simulink model "sm_robot_run_4legs"  (R2025a)
settings: Solver=ode15s  StartTime=0.0  StopTime=t_final  MaxStep=0.01  RelTol=1e-3  AbsTol=1e-4  EnableMultiTasking=on
InitFcn:
  | d2r = pi/180;
  | r2d = 180/pi;
  | if (~exist('t_final'))
  |   sm_robot_run_4legs_param_def_load(bdroot)
  | end
values from neighbouring files (symbols this model uses):
  N = 100    [Extr_Data_Cam_Roller_Curve.m]
  s = sin(q)    [Extr_Data_Cam_Roller_Curve.m]
undefined symbols (not defined in the file or in its folder): Extr_Data_Mesh, l1, L_back, L_stance, M, T_cg, th2, u0, X, Y, Z
libraries: sm_lib x32, nesl_utility x10, fl_lib x5, sm_robot_run_4legs_lib x4, batteryecm_lib x1
(part 1 of 2)
CloseFcn:
  | try,close(h1_sm_robot_run_4legs),end
  | clear h1_sm_robot_run_4legs
  | try,close(h2_sm_robot_run_4legs),end
  | clear h2_sm_robot_run_4legs
  | try,close(h3_sm_robot_run_4legs),end
  | clear h3_sm_robot_run_4legs
  | try,close(h4_sm_robot_run_4legs),end
  | clear h4_sm_robot_run_4legs
  | 
  | 
  | clear simlog_sm_robot_run_4legs
  | clear logsout_sm_robot_run_4legs
Description:
  | Mechatronic Running Robot
  | 
  | Copyright 2012-2025 The MathWorks, Inc.
settings Model: Creator=rhyde  LastModifiedBy=smiller
settings SolverCC: AutoScaleAbsTol=off  MaxConsecutiveZCs=10000  AlgebraicLoopSolver=TrustRegion
settings DataIOCC: MaxDataPoints=10000  SaveFinalState=on  SaveFormat=Array  SignalLoggingSaveFormat=ModelDataLogs  SaveState=on  ReturnWorkspaceOutputs=off  SignalLoggingName=logsout_sm_robot_run_4legs  OutputTimes=[0:0.01:t_final]
settings OptimizationCC: ReuseModelBlockBuffer=off  ExpressionDepthLimit=2147483647.0  InitFltsAndDblsToZero=on  LifeSpan=inf
settings DebuggingCC: SaveWithParameterizedLinksMsg=none  UnderspecifiedInitializationDetection=Classic  MergeDetectMultiDrivingBlocksExec=none  SignalResolutionControl=TryResolveAllWithWarning  SolverPrmCheckMsg=warning  MultiTaskDSMMsg=warning  MultiTaskCondExecSysMsg=none  FcnCallInpInsideContextMsg=warning  UnconnectedInputMsg=warning  UnconnectedOutputMsg=warning  UnconnectedLineMsg=warning  StateNameClashWarn=warning  PregeneratedLibrarySubsystemCodeDiagnostic=none  SFUnexpectedBacktrackingDiag=warning  SFNoUnconditionalDefaultTransitionDiag=warning  SFExecutionAtInitializationDiag=none  ArithmeticOperatorsInVariantConditions=warning
settings HardwareCC: ProdBitPerPointer=32.0  ProdBitPerSizeT=32.0  ProdBitPerPtrDiffT=32.0  ProdLargestAtomicFloat=None  ProdIntDivRoundTo=Undefined  ProdEndianess=Unspecified  ProdWordSize=32.0  ProdHWDeviceType=32-bit Generic
settings ModelReferenceCC: EnableRefExpFcnMdlSchedulingChecks=on  PropagateSignalLabelsOutOfModel=off
settings SFSimCC: SimUseLocalCustomCode=off  SimParseCustomCode=off  CustomCodeUndefinedFunction=UseInterfaceOnly
settings RTWCC: RTWUseLocalCustomCode=off  GPUComputeCapability=3.5  DLArmComputeVersion=19.05
settings CodeAppCC: StateflowObjectComments=on
settings GRTTargetCC: TargetFcnLib=ansi_tfl_tmw.mat  TargetLangStandard=C89/C90 (ANSI)  CombineOutputUpdateFcns=off  GRTInterface=on
settings ConfigComp: CovMetricSettings=dw  CovSaveCumulativeToWorkspaceVar=on  CovSaveSingleToWorkspaceVar=on  CovExternalEMLEnable=off
settings SimscapeCC: SimscapeNormalizeSystem=off  SimscapeLogType=all  SimscapeLogSimulationStatistics=on  SimscapeLogName=simlog_sm_robot_run_4legs  SimscapeLogDataHistory=50000.0
settings ConfigurationSet: Description=SimMechanics 2G
settings DiagnosticsConfigSet: SimMechanicsUnconnectedFramePorts=none  SimMechanicsRigidlyBoundBlock=none
settings ExplorerConfigSet: InternalSimMechanicsExplorerSettings="<ExplorerConfiguration><canonicalview>default</canonicalview><AnimationSetting><BasePlaybackSpeed>1.0</BasePlaybackSpeed><PlaybackSpeedFactor>0.5</PlaybackSpeedFactor></AnimationSetting><TilePanel><TileInfo><Tiles Columns=\"1\" Count=\"1\" Rows=\"1\"><Column Weight=\"1\"/><Row Weight=\"1\"/><Tile Height=\"1\" Width=\"1\" X=\"0\" Y=\"0\"/></Tiles></TileInfo><SceneInfo><SceneViewer><BGColor><R>1</R><G>1</G><B>1</B></BGColor><Camera><DoPerspective>on</DoPerspective><Position><X>9.65055700274290018</X><Y>0.935000000000000053</Y><Z>1.00000000000000089</Z></Position><Center><X>8.79768847079045635</X><Y>0.76135182233306975</Y><Z>0.507596123493896711</Z></Center><Up><X>0</X><Y>1</Y><Z>0</Z></Up><ViewLimDist>1</ViewLimDist><YLim>0.466307658154998583</YLim><XLim>0.552660928183702049</XLim></Camera></SceneViewer></SceneInfo></TilePanel><MechEditorPanel><Cameras><Camera><Id>Camera1</Id><Value><Name>Body</Name><NativeCamera><PositionTrackingFeature>Body_Constraint.Camera.Transform_Camera.F</PositionTrackingFeature><CenterTrackingFeature>Body_Constraint.World_Frame.W</CenterTrackingFeature><UpVectorTrackingFeature>Body_Constraint.World_Frame.W</UpVectorTrackingFeature><CenterTrackingOrigin>off</CenterTrackingOrigin><CenterTrackingDirection>-Z</CenterTrackingDirection><UpVectorTrackingDirection>+Y</UpVectorTrackingDirection></NativeCamera></Value></Camera><Camera><Id>Camera2</Id><Value><Name>Body_Iso</Name><NativeCamera><PositionTrackingFeature>Body_Constraint.Camera.Transform_Camera_BodyIso.F</PositionTrackingFeature><CenterTrackingFeature>Body_Constraint.Camera.Transform_Camera_BodyIso_Aim.F</CenterTrackingFeature><UpVectorTrackingFeature>Body_Constraint.World_Frame.W</UpVectorTrackingFeature><CenterTrackingOrigin>off</CenterTrackingOrigin><CenterTrackingDirection>-Z</CenterTrackingDirection><UpVectorTrackingDirection>+Y</UpVectorTrackingDirection></NativeCamera></Value></Camera></Cameras><GfxPanelCameraMap><MapElement CameraMLId=\"Camera2\" GfxPanelIndex=\"0\"/></GfxPanelCameraMap><VideoCreator><PlaybackSpeedRatio>1.0</PlaybackSpeedRatio><FrameRate>30</FrameRate><VideoFormat>Motion JPEG AVI</VideoFormat><FrameSize>auto</FrameSize></VideoCreator></MechEditorPanel></ExplorerConfiguration>"

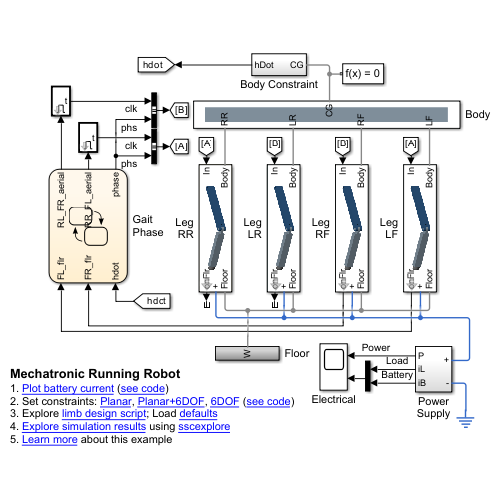
[thumbnail: Simulink's stored preview of the top-level diagram]
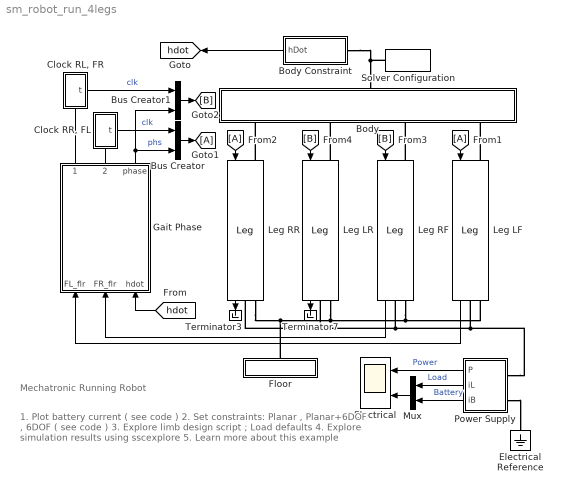
== system sm_robot_run_4legs ==
  note: Mechatronic Running Robot
  note: 1. Plot battery current ( see code )
      | 2. Set constraints: Planar , Planar+6DOF , 6DOF ( see code )
      | 3. Explore limb design script ; Load defaults
      | 4. Explore simulation results using sscexplore
      | 5. Learn more about this example
  Body : Subsystem  Tag=CustomStyle
      mask Display: image('sm_robot_run_body_IMAGE.png')
  Body Constraint : Subsystem
  Bus Creator : BusCreator  Inputs=2
  Bus Creator1 : BusCreator  Inputs=2
  "Clock RL, FR" : Subsystem  TreatAsAtomicUnit=on  mask{t0=0}
      mask prompts: t0 "Initial local time"
  "Clock RR, FL" : Subsystem  TreatAsAtomicUnit=on  mask{t0=3*T_cg/4}
      mask prompts: t0 "Initial local time"
  Electrical : Scope  NumInputPorts=2
      settings: ActiveDisplayYMinimum=-181.58066  ActiveDisplayYMaximum=525.06229
  Electrical Reference : fl_lib/Electrical/Electrical Elements/Electrical Reference
  Floor : Subsystem
  From1 : From
  From2 : From
  Gait Phase : Stateflow chart  Tag=PublishSubsystem  TreatAsAtomicUnit=on
  Goto1 : Goto
  Leg LF : sm_robot_run_4legs_lib/Leg  Tag=PublishSubsystemCustomStyle  leg_type=Front Left  leg_width=0.1*l1  th1_0=d2r*u_th(find(t_th > 3*T_cg/4,1))  th2_0=-50*d2r+th2  th1_dot_0=-d2r*u_w(find(t_th > 3*T_cg/4,1))  x0=L_back  popup_contact_model=Planar
  Leg LR : sm_robot_run_4legs_lib/Leg  Tag=CustomStyle  leg_type=Rear Left  leg_width=0.1*l1  th1_0=th1_0  th2_0=th2_0  th1_dot_0=u0/L_stance  x0=0  popup_contact_model=Planar
  Leg RF : sm_robot_run_4legs_lib/Leg  Tag=CustomStyle  leg_type=Front Right  leg_width=0.1*l1  th1_0=th1_0  th2_0=th2_0  th1_dot_0=u0/L_stance  x0=L_back  popup_contact_model=Planar
  Leg RR : sm_robot_run_4legs_lib/Leg  Tag=CustomStyle  leg_type=Rear Right  leg_width=0.1*l1  th1_0=d2r*u_th(find(t_th > 3*T_cg/4,1))  th2_0=-50*d2r+th2  th1_dot_0=-d2r*u_w(find(t_th > 3*T_cg/4,1))  x0=0  popup_contact_model=Planar
  Mux : Mux  Inputs=2
  Power Supply : Subsystem  Tag=PublishSubsystem
  Solver Configuration : nesl_utility/Solver Configuration  PhysicalDomain=network_engine_domain  SubClassName=solver  LeftPortType=input  RightPortType=generic  Tones=[]  Harmonics=[]  SimulateNoise=off  Profile=off  UseLocalSampling=off  EnableSwitchedLinearOptims=on  FrequencyDomain=off  UseCCode=off  RelTol=0.001  AbsTol=1e-06  MinStep=1e-09  ToWorkspace=off  RevertToSquareIcSolve=off  NumHomotopyIterations=100  PhasorMode=off  PhasorModeNumHarmonics=1  ConsistencySolver=NEWTON_FTOL  IndexReductionMethod=DerivativeReplacement  DoDC=off  ResidualTolerance=1e-9  ConsistencyTolSource=GLOBAL  ConsistencyAbsTol=0.001  ConsistencyRelTol=0.001  ConsistencyTolFactor=0.001  UseLocalSolver=off  LocalSolverChoice=NE_BACKWARD_EULER_ADVANCER  ResolveIndetEquations=on  FunctionEvalNumThread=1  LocalSolverSampleTime=.001  DoFixedCost=off  MaxNonlinIter=12  MaxModeIter=2  ComputeImpulses=off  ImpulseIterations=2  LinearAlgebra=Sparse  LinearAlgebraNumThread=0  EquationFormulation=NE_TIME_EF  DelaysMemoryBudget=1024  AutomaticFiltering=on  FilteringTimeConstant=0.001  PartitionStorageMethod=AS_NEEDED  PartitionMemoryBudget=1024  PartitionMethod=FAST  MultibodyUseLocalSolver=off  MultibodyLocalSolverChoice=ODE1  MultibodyLocalSolverSampleTime=0.001
  Terminator3 : Terminator
  Terminator7 : Terminator
  tag scope: hdot=global
  wires:
  [hdot] -> Gait Phase/3(hdot)
  Leg RR/1 -> Terminator3/1
  Leg LF/1 -> Gait Phase/1(FL_flr)
  Leg LR/1 -> Terminator7/1
  Gait Phase/1(RL_FR_aerial) -> "Clock RL, FR"/Enable
  Gait Phase/2(RR_FL_aerial) -> "Clock RR, FL"/Enable
  "Clock RR, FL"/1(t) -> Bus Creator/1  "clk"
  Leg RF/1 -> Gait Phase/2(FR_flr)
  Power Supply/2(iL) -> Mux/1  "Load"
  Power Supply/1(P) -> Electrical/1  "Power"
  Bus Creator/1 -> Goto1/1
  Bus Creator1/1 -> [B]
  "Clock RL, FR"/1(t) -> Bus Creator1/1  "clk"
  Gait Phase/3(phase) -> Bus Creator1/2, Bus Creator/2  "phs"
  From1/1 -> Leg LF/1
  From2/1 -> Leg RR/1
  [B] -> Leg RF/1
  [B] -> Leg LR/1
  Body Constraint/1(hDot) -> [hdot]
  Mux/1 -> Electrical/2
  Power Supply/3(iB) -> Mux/2  "Battery"
  connections:
  Body Constraint/LConn1 -- Solver Configuration/RConn1 -- Body/RConn1
  Power Supply/LConn2 -- Electrical Reference/LConn1
  Power Supply/LConn1 -- Leg RR/RConn1 -- Leg LR/RConn1 -- Leg RF/RConn1 -- Leg LF/RConn1
  Leg LF/LConn1 -- Body/LConn4
  Leg RF/LConn1 -- Body/LConn3
  Leg LR/LConn1 -- Body/LConn2
  Leg RR/LConn1 -- Body/LConn1
  Floor/RConn1 -- Leg LF/RConn2 -- Leg RF/RConn2 -- Leg LR/RConn2 -- Leg RR/RConn2

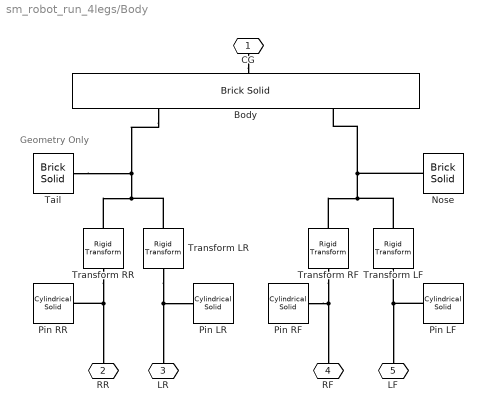
== system sm_robot_run_4legs/Body ==
  note: Geometry Only
  Body : sm_lib/Body Elements/Brick Solid  BrickDimensions=[1 0.1 0.1]*L_back  BrickDimensionsUnits=m  ExportEntireGeometry=off  InertiaType=Custom  BasedOnType=Density  Density=1000  DensityUnits=kg/m^3  Mass=M*2  MassUnits=kg  CenterOfMass=[0 0 0]  CenterOfMassUnits=m  MomentsOfInertia=[1 1 1]*(1/12)*2*M*L_back^2*100  MomentsOfInertiaUnits=kg*m^2  ProductsOfInertia=[1 1 1]*0  ProductsOfInertiaUnits=kg*m^2  GraphicType=FromGeometry  MarkerShape=Sphere  MarkerSize=10  GraphicVisPropType=SimpleVisualProperties  GraphicDiffuseColor=[164 184 200]/255  GraphicOpacity=1.0  GraphicSpecularColor=[0.5 0.5 0.5 1.0]  GraphicAmbientColor=[0.15 0.15 0.15 1.0]  GraphicEmissiveColor=[0.0 0.0 0.0 1.0]  GraphicShininess=75  DoExposeReferenceFrame=on  SerializedFrames=<Frames><Frame><Id>Frame1</Id><Value><Name>B</Name><Origin><Source>GeometricFeature</Source><FeatureName>-x surface</FeatureName></Origin><PrimaryAxis><DefinedDirection>+Z</DefinedDirection><Source>ReferenceFrame</Source><SourceDirection>+Z</SourceDirection><FeatureName></FeatureName></PrimaryAxis><SecondaryAxis><DefinedDirection>+X</DefinedDirection><Source>ReferenceFrame</Source><SourceDirection>+X</SourceDirection><FeatureName></FeatureName></SecondaryAxis></Value></Frame><Frame><Id>Frame2</Id><Value><Name>F</Name><Origin><Source>GeometricFeature</Source><FeatureName>+x surface</FeatureName></Origin><PrimaryAxis><DefinedDirection>+Z</DefinedDirection><Source>ReferenceFrame</Source><SourceDirection>+Z</SourceDirection><FeatureName></FeatureName></PrimaryAxis><SecondaryAxis><DefinedDirection>+X</DefinedDirection><Source>ReferenceFrame</Source><SourceDirection>+X</SourceDirection><FeatureName></FeatureName></SecondaryAxis></Value></Frame></Frames>
  Nose : sm_lib/Body Elements/Brick Solid  BrickDimensions=[0.05 0.1 0.1]*L_back  BrickDimensionsUnits=m  ExportEntireGeometry=off  InertiaType=CalculateFromGeometry  BasedOnType=Density  Density=0  DensityUnits=kg/m^3  Mass=1  MassUnits=kg  CenterOfMass=[0 0 0]  CenterOfMassUnits=m  MomentsOfInertia=[1 1 1]  MomentsOfInertiaUnits=kg*m^2  ProductsOfInertia=[1 1 1]  ProductsOfInertiaUnits=kg*m^2  GraphicType=FromGeometry  MarkerShape=Sphere  MarkerSize=10  GraphicVisPropType=SimpleVisualProperties  GraphicDiffuseColor=[164 184 200]/255  GraphicOpacity=1.0  GraphicSpecularColor=[0.5 0.5 0.5 1.0]  GraphicAmbientColor=[0.15 0.15 0.15 1.0]  GraphicEmissiveColor=[0.0 0.0 0.0 1.0]  GraphicShininess=75  DoExposeReferenceFrame=off  SerializedFrames=<Frames><Frame><Id>Frame1</Id><Value><Name>B</Name><Origin><Source>GeometricFeature</Source><FeatureName>-x surface</FeatureName></Origin><PrimaryAxis><DefinedDirection>+Z</DefinedDirection><Source>ReferenceFrame</Source><SourceDirection>+Z</SourceDirection><FeatureName></FeatureName></PrimaryAxis><SecondaryAxis><DefinedDirection>+X</DefinedDirection><Source>ReferenceFrame</Source><SourceDirection>+X</SourceDirection><FeatureName></FeatureName></SecondaryAxis></Value></Frame></Frames>
  Pin LF : sm_lib/Body Elements/Cylindrical Solid  CylinderRadius=0.025*l1  CylinderRadiusUnits=m  CylinderLength=0.1*l1  CylinderLengthUnits=m  ExportEntireGeometry=off  InertiaType=CalculateFromGeometry  BasedOnType=Density  Density=0  DensityUnits=kg/m^3  Mass=1  MassUnits=kg  CenterOfMass=[0 0 0]  CenterOfMassUnits=m  MomentsOfInertia=[1 1 1]  MomentsOfInertiaUnits=kg*m^2  ProductsOfInertia=[1 1 1]  ProductsOfInertiaUnits=kg*m^2  GraphicType=FromGeometry  MarkerShape=Sphere  MarkerSize=10  GraphicVisPropType=SimpleVisualProperties  GraphicDiffuseColor=[164 184 200]/255  GraphicOpacity=1.0  GraphicSpecularColor=[0.5 0.5 0.5 1.0]  GraphicAmbientColor=[0.15 0.15 0.15 1.0]  GraphicEmissiveColor=[0.0 0.0 0.0 1.0]  GraphicShininess=75  DoExposeReferenceFrame=off  SerializedFrames=<Frames><Frame><Id>Frame1</Id><Value><Name>F</Name><Origin><Source>GeometricFeature</Source><FeatureName>top surface</FeatureName></Origin><PrimaryAxis><DefinedDirection>+Z</DefinedDirection><Source>ReferenceFrame</Source><SourceDirection>+Z</SourceDirection><FeatureName></FeatureName></PrimaryAxis><SecondaryAxis><DefinedDirection>+X</DefinedDirection><Source>ReferenceFrame</Source><SourceDirection>+X</SourceDirection><FeatureName></FeatureName></SecondaryAxis></Value></Frame><Frame><Id>Frame2</Id><Value><Name>B</Name><Origin><Source>GeometricFeature</Source><FeatureName>bottom surface</FeatureName></Origin><PrimaryAxis><DefinedDirection>+Z</DefinedDirection><Source>ReferenceFrame</Source><SourceDirection>+Z</SourceDirection><FeatureName></FeatureName></PrimaryAxis><SecondaryAxis><DefinedDirection>+X</DefinedDirection><Source>ReferenceFrame</Source><SourceDirection>+X</SourceDirection><FeatureName></FeatureName></SecondaryAxis></Value></Frame></Frames>
  Pin LR : sm_lib/Body Elements/Cylindrical Solid  CylinderRadius=0.025*l1  CylinderRadiusUnits=m  CylinderLength=0.1*l1  CylinderLengthUnits=m  ExportEntireGeometry=off  InertiaType=CalculateFromGeometry  BasedOnType=Density  Density=0  DensityUnits=kg/m^3  Mass=1  MassUnits=kg  CenterOfMass=[0 0 0]  CenterOfMassUnits=m  MomentsOfInertia=[1 1 1]  MomentsOfInertiaUnits=kg*m^2  ProductsOfInertia=[1 1 1]  ProductsOfInertiaUnits=kg*m^2  GraphicType=FromGeometry  MarkerShape=Sphere  MarkerSize=10  GraphicVisPropType=SimpleVisualProperties  GraphicDiffuseColor=[164 184 200]/255  GraphicOpacity=1.0  GraphicSpecularColor=[0.5 0.5 0.5 1.0]  GraphicAmbientColor=[0.15 0.15 0.15 1.0]  GraphicEmissiveColor=[0.0 0.0 0.0 1.0]  GraphicShininess=75  DoExposeReferenceFrame=off  SerializedFrames=<Frames><Frame><Id>Frame1</Id><Value><Name>F</Name><Origin><Source>GeometricFeature</Source><FeatureName>top surface</FeatureName></Origin><PrimaryAxis><DefinedDirection>+Z</DefinedDirection><Source>ReferenceFrame</Source><SourceDirection>+Z</SourceDirection><FeatureName></FeatureName></PrimaryAxis><SecondaryAxis><DefinedDirection>+X</DefinedDirection><Source>ReferenceFrame</Source><SourceDirection>+X</SourceDirection><FeatureName></FeatureName></SecondaryAxis></Value></Frame><Frame><Id>Frame2</Id><Value><Name>B</Name><Origin><Source>GeometricFeature</Source><FeatureName>bottom surface</FeatureName></Origin><PrimaryAxis><DefinedDirection>+Z</DefinedDirection><Source>ReferenceFrame</Source><SourceDirection>+Z</SourceDirection><FeatureName></FeatureName></PrimaryAxis><SecondaryAxis><DefinedDirection>+X</DefinedDirection><Source>ReferenceFrame</Source><SourceDirection>+X</SourceDirection><FeatureName></FeatureName></SecondaryAxis></Value></Frame></Frames>
  Pin RF : sm_lib/Body Elements/Cylindrical Solid  CylinderRadius=0.025*l1  CylinderRadiusUnits=m  CylinderLength=0.1*l1  CylinderLengthUnits=m  ExportEntireGeometry=off  InertiaType=CalculateFromGeometry  BasedOnType=Density  Density=0  DensityUnits=kg/m^3  Mass=1  MassUnits=kg  CenterOfMass=[0 0 0]  CenterOfMassUnits=m  MomentsOfInertia=[1 1 1]  MomentsOfInertiaUnits=kg*m^2  ProductsOfInertia=[1 1 1]  ProductsOfInertiaUnits=kg*m^2  GraphicType=FromGeometry  MarkerShape=Sphere  MarkerSize=10  GraphicVisPropType=SimpleVisualProperties  GraphicDiffuseColor=[164 184 200]/255  GraphicOpacity=1.0  GraphicSpecularColor=[0.5 0.5 0.5 1.0]  GraphicAmbientColor=[0.15 0.15 0.15 1.0]  GraphicEmissiveColor=[0.0 0.0 0.0 1.0]  GraphicShininess=75  DoExposeReferenceFrame=off  SerializedFrames=<Frames><Frame><Id>Frame1</Id><Value><Name>F</Name><Origin><Source>GeometricFeature</Source><FeatureName>top surface</FeatureName></Origin><PrimaryAxis><DefinedDirection>+Z</DefinedDirection><Source>ReferenceFrame</Source><SourceDirection>+Z</SourceDirection><FeatureName></FeatureName></PrimaryAxis><SecondaryAxis><DefinedDirection>+X</DefinedDirection><Source>ReferenceFrame</Source><SourceDirection>+X</SourceDirection><FeatureName></FeatureName></SecondaryAxis></Value></Frame><Frame><Id>Frame2</Id><Value><Name>B</Name><Origin><Source>GeometricFeature</Source><FeatureName>bottom surface</FeatureName></Origin><PrimaryAxis><DefinedDirection>+Z</DefinedDirection><Source>ReferenceFrame</Source><SourceDirection>+Z</SourceDirection><FeatureName></FeatureName></PrimaryAxis><SecondaryAxis><DefinedDirection>+X</DefinedDirection><Source>ReferenceFrame</Source><SourceDirection>+X</SourceDirection><FeatureName></FeatureName></SecondaryAxis></Value></Frame></Frames>
  Pin RR : sm_lib/Body Elements/Cylindrical Solid  CylinderRadius=0.025*l1  CylinderRadiusUnits=m  CylinderLength=0.1*l1  CylinderLengthUnits=m  ExportEntireGeometry=off  InertiaType=CalculateFromGeometry  BasedOnType=Density  Density=0  DensityUnits=kg/m^3  Mass=1  MassUnits=kg  CenterOfMass=[0 0 0]  CenterOfMassUnits=m  MomentsOfInertia=[1 1 1]  MomentsOfInertiaUnits=kg*m^2  ProductsOfInertia=[1 1 1]  ProductsOfInertiaUnits=kg*m^2  GraphicType=FromGeometry  MarkerShape=Sphere  MarkerSize=10  GraphicVisPropType=SimpleVisualProperties  GraphicDiffuseColor=[164 184 200]/255  GraphicOpacity=1.0  GraphicSpecularColor=[0.5 0.5 0.5 1.0]  GraphicAmbientColor=[0.15 0.15 0.15 1.0]  GraphicEmissiveColor=[0.0 0.0 0.0 1.0]  GraphicShininess=75  DoExposeReferenceFrame=off  SerializedFrames=<Frames><Frame><Id>Frame1</Id><Value><Name>F</Name><Origin><Source>GeometricFeature</Source><FeatureName>top surface</FeatureName></Origin><PrimaryAxis><DefinedDirection>+Z</DefinedDirection><Source>ReferenceFrame</Source><SourceDirection>+Z</SourceDirection><FeatureName></FeatureName></PrimaryAxis><SecondaryAxis><DefinedDirection>+X</DefinedDirection><Source>ReferenceFrame</Source><SourceDirection>+X</SourceDirection><FeatureName></FeatureName></SecondaryAxis></Value></Frame><Frame><Id>Frame2</Id><Value><Name>B</Name><Origin><Source>GeometricFeature</Source><FeatureName>bottom surface</FeatureName></Origin><PrimaryAxis><DefinedDirection>+Z</DefinedDirection><Source>ReferenceFrame</Source><SourceDirection>+Z</SourceDirection><FeatureName></FeatureName></PrimaryAxis><SecondaryAxis><DefinedDirection>+X</DefinedDirection><Source>ReferenceFrame</Source><SourceDirection>+X</SourceDirection><FeatureName></FeatureName></SecondaryAxis></Value></Frame></Frames>
  Tail : sm_lib/Body Elements/Brick Solid  BrickDimensions=[0.05 0.1 0.1]*L_back  BrickDimensionsUnits=m  ExportEntireGeometry=off  InertiaType=CalculateFromGeometry  BasedOnType=Density  Density=0  DensityUnits=kg/m^3  Mass=1  MassUnits=kg  CenterOfMass=[0 0 0]  CenterOfMassUnits=m  MomentsOfInertia=[1 1 1]  MomentsOfInertiaUnits=kg*m^2  ProductsOfInertia=[1 1 1]  ProductsOfInertiaUnits=kg*m^2  GraphicType=FromGeometry  MarkerShape=Sphere  MarkerSize=10  GraphicVisPropType=SimpleVisualProperties  GraphicDiffuseColor=[164 184 200]/255  GraphicOpacity=1.0  GraphicSpecularColor=[0.5 0.5 0.5 1.0]  GraphicAmbientColor=[0.15 0.15 0.15 1.0]  GraphicEmissiveColor=[0.0 0.0 0.0 1.0]  GraphicShininess=75  DoExposeReferenceFrame=off  SerializedFrames=<Frames><Frame><Id>Frame1</Id><Value><Name>F</Name><Origin><Source>GeometricFeature</Source><FeatureName>+x surface</FeatureName></Origin><PrimaryAxis><DefinedDirection>+Z</DefinedDirection><Source>ReferenceFrame</Source><SourceDirection>+Z</SourceDirection><FeatureName></FeatureName></PrimaryAxis><SecondaryAxis><DefinedDirection>+X</DefinedDirection><Source>ReferenceFrame</Source><SourceDirection>+X</SourceDirection><FeatureName></FeatureName></SecondaryAxis></Value></Frame></Frames>
  Transform LF : sm_lib/Frames and Transforms/Rigid Transform  RotationMethod=None  FollAlignAxisA=+X  BaseAlignAxisA=+Y  FollAlignAxisB=+Y  BaseAlignAxisB=+Z  RotationStandardAxis=+Z  RotationAngle=0.0  RotationAngleUnits=deg  RotationArbitraryAxis=[0 0 1]  RotationSequenceAxes=FollowerAxes  RotationSequence=XYX  RotationSequenceAngles=[0 0 0]  RotationSequenceAnglesUnits=deg  RotationMatrix=[1 0 0; 0 1 0; 0 0 1]  Quaternion=[1 0 0 0]  TranslationMethod=StandardAxis  TranslationCartesianOffset=[0 0 0]  TranslationCartesianOffsetUnits=m  TranslationStandardAxis=+Z  TranslationStandardOffset=0.1*L_back/2  TranslationStandardOffsetUnits=m  TranslationROffset=0  TranslationROffsetUnits=m  TranslationThetaOffset=0  TranslationThetaOffsetUnits=deg  TranslationZOffset=0  TranslationZOffsetUnits=m
  Transform LR : sm_lib/Frames and Transforms/Rigid Transform  RotationMethod=None  FollAlignAxisA=+X  BaseAlignAxisA=+Y  FollAlignAxisB=+Y  BaseAlignAxisB=+Z  RotationStandardAxis=+Z  RotationAngle=0.0  RotationAngleUnits=deg  RotationArbitraryAxis=[0 0 1]  RotationSequenceAxes=FollowerAxes  RotationSequence=XYX  RotationSequenceAngles=[0 0 0]  RotationSequenceAnglesUnits=deg  RotationMatrix=[1 0 0; 0 1 0; 0 0 1]  Quaternion=[1 0 0 0]  TranslationMethod=StandardAxis  TranslationCartesianOffset=[0 0 0]  TranslationCartesianOffsetUnits=m  TranslationStandardAxis=+Z  TranslationStandardOffset=0.1*L_back/2  TranslationStandardOffsetUnits=m  TranslationROffset=0  TranslationROffsetUnits=m  TranslationThetaOffset=0  TranslationThetaOffsetUnits=deg  TranslationZOffset=0  TranslationZOffsetUnits=m
  Transform RF : sm_lib/Frames and Transforms/Rigid Transform  RotationMethod=None  FollAlignAxisA=+X  BaseAlignAxisA=+Y  FollAlignAxisB=+Y  BaseAlignAxisB=+Z  RotationStandardAxis=+Z  RotationAngle=0.0  RotationAngleUnits=deg  RotationArbitraryAxis=[0 0 1]  RotationSequenceAxes=FollowerAxes  RotationSequence=XYX  RotationSequenceAngles=[0 0 0]  RotationSequenceAnglesUnits=deg  RotationMatrix=[1 0 0; 0 1 0; 0 0 1]  Quaternion=[1 0 0 0]  TranslationMethod=StandardAxis  TranslationCartesianOffset=[0 0 0]  TranslationCartesianOffsetUnits=m  TranslationStandardAxis=+Z  TranslationStandardOffset=0.1*L_back/2  TranslationStandardOffsetUnits=m  TranslationROffset=0  TranslationROffsetUnits=m  TranslationThetaOffset=0  TranslationThetaOffsetUnits=deg  TranslationZOffset=0  TranslationZOffsetUnits=m
  Transform RR : sm_lib/Frames and Transforms/Rigid Transform  RotationMethod=None  FollAlignAxisA=+X  BaseAlignAxisA=+Y  FollAlignAxisB=+Y  BaseAlignAxisB=+Z  RotationStandardAxis=+Z  RotationAngle=0.0  RotationAngleUnits=deg  RotationArbitraryAxis=[0 0 1]  RotationSequenceAxes=FollowerAxes  RotationSequence=XYX  RotationSequenceAngles=[0 0 0]  RotationSequenceAnglesUnits=deg  RotationMatrix=[1 0 0; 0 1 0; 0 0 1]  Quaternion=[1 0 0 0]  TranslationMethod=StandardAxis  TranslationCartesianOffset=[0 0 0]  TranslationCartesianOffsetUnits=m  TranslationStandardAxis=+Z  TranslationStandardOffset=0.1*L_back/2  TranslationStandardOffsetUnits=m  TranslationROffset=0  TranslationROffsetUnits=m  TranslationThetaOffset=0  TranslationThetaOffsetUnits=deg  TranslationZOffset=0  TranslationZOffsetUnits=m
  CG : PMIOPort  Side=Right
  RR : PMIOPort  Port=2  Side=Left
  LR : PMIOPort  Port=3  Side=Left
  RF : PMIOPort  Port=4  Side=Left
  LF : PMIOPort  Port=5  Side=Left
  connections:
  Pin LF/RConn1 -- LF/RConn1 -- Transform LF/RConn1
  CG/RConn1 -- Body/RConn1
  Transform LF/LConn1 -- Transform RF/RConn1 -- Body/LConn2 -- Nose/LConn1
  Transform RF/LConn1 -- RF/RConn1 -- Pin RF/LConn1
  Body/LConn1 -- Tail/LConn1 -- Transform LR/LConn1 -- Transform RR/RConn1
  Transform RR/LConn1 -- Pin RR/LConn1 -- RR/RConn1
  Transform LR/RConn1 -- LR/RConn1 -- Pin LR/RConn1

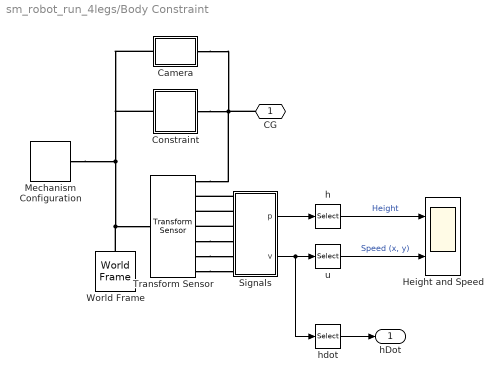
== system sm_robot_run_4legs/Body Constraint ==
  Camera : Subsystem
  Constraint : Subsystem  Variant=on  VariantControlMode=label  VariantControl=Variant1  LabelModeActiveChoice=Planar
      settings: AttributesFormatString=%<ActiveVariant>
      mask Display: disp(' ')
  Height and Speed : Scope  NumInputPorts=2
      settings: ActiveDisplayYMinimum=0.80791  ActiveDisplayYMaximum=1.22878
  Mechanism Configuration : sm_lib/Utilities/Mechanism Configuration  UniformGravity=Constant  GravityVector=[0 -9.81 0]  GravityVectorUnits=m/s^2  LinearizationDelta=0.001  JointModeTransitionNonlinearIterations=2
  Signals : Subsystem
  Transform Sensor : sm_lib/Frames and Transforms/Transform Sensor  MeasurementFrame=World  RotationSequence=XYX  SenseAngle=off  SenseAxis=off  SenseQ=off  SenseR=off  SenseRotationSequence=off  SenseOmegaX=off  SenseOmegaY=off  SenseOmegaZ=off  SenseOmega=off  SenseQDot=off  SenseRDot=off  SenseRotationSequenceDot=off  SenseAlphaX=off  SenseAlphaY=off  SenseAlphaZ=off  SenseAlpha=off  SenseQDDot=off  SenseRDDot=off  SenseX=on  SenseY=on  SenseZ=on  SenseXYZ=off  SenseRad=off  SenseAzim=off  SenseDist=off  SenseInc=off  SenseXDot=on  SenseYDot=on  SenseZDot=on  SenseXYZDot=off  SenseRadDot=off  SenseAzimDot=off  SenseDistDot=off  SenseIncDot=off  SenseXDDot=off  SenseYDDot=off  SenseZDDot=off  SenseXYZDDot=off  SenseRadDDot=off  SenseAzimDDot=off  SenseDistDDot=off  SenseIncDDot=off
  World Frame : sm_lib/Frames and Transforms/World Frame
  h : Selector  InputPortWidth=3  IndexOptions=Index vector (dialog)  Indices=2  OutputSizes=1
  hdot : Selector  InputPortWidth=3  IndexOptions=Index vector (dialog)  Indices=2  OutputSizes=1
  u : Selector  InputPortWidth=3  IndexOptions=Index vector (dialog)  Indices=[1 2]  OutputSizes=1
  CG : PMIOPort  Side=Left
  hDot : Outport  VectorParamsAs1DForOutWhenUnconnected=off
  wires:
  Signals/2(v) -> hdot/1, u/1
  Signals/1(p) -> h/1
  hdot/1 -> hDot/1
  u/1 -> Height and Speed/2  "Speed (x, y)"
  h/1 -> Height and Speed/1  "Height"
  connections:
  Transform Sensor/RConn6 -- Signals/LConn5
  Signals/LConn1 -- Transform Sensor/RConn2
  Signals/LConn3 -- Transform Sensor/RConn4
  Transform Sensor/RConn7 -- Signals/LConn6
  Transform Sensor/RConn5 -- Signals/LConn4
  Signals/LConn2 -- Transform Sensor/RConn3
  CG/RConn1 -- Constraint/RConn1 -- Camera/RConn1 -- Transform Sensor/RConn1
  Mechanism Configuration/RConn1 -- Constraint/LConn1 -- Camera/LConn1 -- World Frame/RConn1 -- Transform Sensor/LConn1

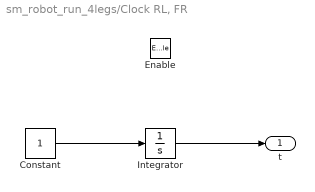
== system sm_robot_run_4legs/Clock RL, FR ==
  Enable : EnablePort  StatesWhenEnabling=reset
  Constant : Constant
  Integrator : Integrator  InitialCondition=t0
  t : Outport  OutputWhenDisabled=reset  InitialOutput=[0]  VectorParamsAs1DForOutWhenUnconnected=off
  wires:
  Integrator/1 -> t/1
  Constant/1 -> Integrator/1

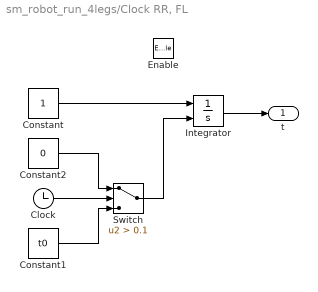
== system sm_robot_run_4legs/Clock RR, FL ==
  Enable : EnablePort  StatesWhenEnabling=reset
  Clock : Clock
  Constant : Constant
  Constant1 : Constant  Value=t0
  Constant2 : Constant  Value=0
  Integrator : Integrator  InitialConditionSource=external  InitialCondition=t0
  Switch : Switch  Criteria=u2 > Threshold  Threshold=0.1  SaturateOnIntegerOverflow=off  InputSameDT=off
  t : Outport  OutputWhenDisabled=reset  InitialOutput=0  VectorParamsAs1DForOutWhenUnconnected=off
  wires:
  Constant/1 -> Integrator/1
  Integrator/1 -> t/1
  Switch/1 -> Integrator/2
  Constant1/1 -> Switch/3
  Constant2/1 -> Switch/1
  Clock/1 -> Switch/2

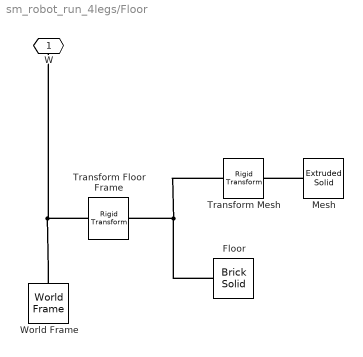
== system sm_robot_run_4legs/Floor ==
  Floor : sm_lib/Body Elements/Brick Solid  BrickDimensions=[100 0.05 1]  BrickDimensionsUnits=m  ExportEntireGeometry=off  InertiaType=CalculateFromGeometry  BasedOnType=Density  Density=1000  DensityUnits=kg/m^3  Mass=1  MassUnits=kg  CenterOfMass=[0 0 0]  CenterOfMassUnits=m  MomentsOfInertia=[1 1 1]  MomentsOfInertiaUnits=kg*m^2  ProductsOfInertia=[1 1 1]  ProductsOfInertiaUnits=kg*m^2  GraphicType=FromGeometry  MarkerShape=Sphere  MarkerSize=10  GraphicVisPropType=SimpleVisualProperties  GraphicDiffuseColor=[0.5 0.5 0.5]  GraphicOpacity=1.0  GraphicSpecularColor=[0.5 0.5 0.5 1.0]  GraphicAmbientColor=[0.15 0.15 0.15 1.0]  GraphicEmissiveColor=[0.0 0.0 0.0 1.0]  GraphicShininess=75  DoExposeReferenceFrame=on  SerializedFrames=<Frames/>
  Mesh : sm_lib/Body Elements/Extruded Solid  ExtrusionType=General  PolygonNumSides=3  PolygonOuterRadius=1  PolygonOuterRadiusUnits=m  ExportEntireGeometry=off  ExtrusionCrossSection=Extr_Data_Mesh(100,1,100,1,0.9,0.9)  ExtrusionCrossSectionUnits=m  ExportConvexHullGeometry=off  ExtrusionLength=0.055  ExtrusionLengthUnits=m  InertiaType=CalculateFromGeometry  BasedOnType=Density  Density=1000  DensityUnits=kg/m^3  Mass=1  MassUnits=kg  CenterOfMass=[0 0 0]  CenterOfMassUnits=m  MomentsOfInertia=[1 1 1]  MomentsOfInertiaUnits=kg*m^2  ProductsOfInertia=[1 1 1]  ProductsOfInertiaUnits=kg*m^2  GraphicType=FromGeometry  MarkerShape=Sphere  MarkerSize=10  GraphicVisPropType=SimpleVisualProperties  GraphicDiffuseColor=[1.0 1.0 1.0]  GraphicOpacity=1.0  GraphicSpecularColor=[0.5 0.5 0.5 1.0]  GraphicAmbientColor=[0.15 0.15 0.15 1.0]  GraphicEmissiveColor=[0.0 0.0 0.0 1.0]  GraphicShininess=75  DoExposeReferenceFrame=on  SerializedFrames=<Frames/>
  Transform Floor Frame : sm_lib/Frames and Transforms/Rigid Transform  RotationMethod=None  FollAlignAxisA=+X  BaseAlignAxisA=+Y  FollAlignAxisB=+Y  BaseAlignAxisB=+Z  RotationStandardAxis=+X  RotationAngle=-90  RotationAngleUnits=deg  RotationArbitraryAxis=[0 0 1]  RotationSequenceAxes=FollowerAxes  RotationSequence=XYX  RotationSequenceAngles=[0 0 0]  RotationSequenceAnglesUnits=deg  RotationMatrix=[1 0 0; 0 1 0; 0 0 1]  Quaternion=[1 0 0 0]  TranslationMethod=StandardAxis  TranslationCartesianOffset=[0 0 0]  TranslationCartesianOffsetUnits=m  TranslationStandardAxis=-Y  TranslationStandardOffset=0.056/2  TranslationStandardOffsetUnits=m  TranslationROffset=0  TranslationROffsetUnits=m  TranslationThetaOffset=0  TranslationThetaOffsetUnits=deg  TranslationZOffset=0  TranslationZOffsetUnits=m
  Transform Mesh : sm_lib/Frames and Transforms/Rigid Transform  RotationMethod=StandardAxis  FollAlignAxisA=+X  BaseAlignAxisA=+Y  FollAlignAxisB=+Y  BaseAlignAxisB=+Z  RotationStandardAxis=-X  RotationAngle=90  RotationAngleUnits=deg  RotationArbitraryAxis=[0 0 1]  RotationSequenceAxes=FollowerAxes  RotationSequence=XYX  RotationSequenceAngles=[0 0 0]  RotationSequenceAnglesUnits=deg  RotationMatrix=[1 0 0; 0 1 0; 0 0 1]  Quaternion=[1 0 0 0]  TranslationMethod=None  TranslationCartesianOffset=[0 0 0]  TranslationCartesianOffsetUnits=m  TranslationStandardAxis=+Z  TranslationStandardOffset=0  TranslationStandardOffsetUnits=m  TranslationROffset=0  TranslationROffsetUnits=m  TranslationThetaOffset=0  TranslationThetaOffsetUnits=deg  TranslationZOffset=0  TranslationZOffsetUnits=m
  World Frame : sm_lib/Frames and Transforms/World Frame
  W : PMIOPort  Side=Right
  connections:
  Mesh/RConn1 -- Transform Mesh/RConn1
  Floor/RConn1 -- Transform Mesh/LConn1 -- Transform Floor Frame/RConn1
  Transform Floor Frame/LConn1 -- W/RConn1 -- World Frame/RConn1

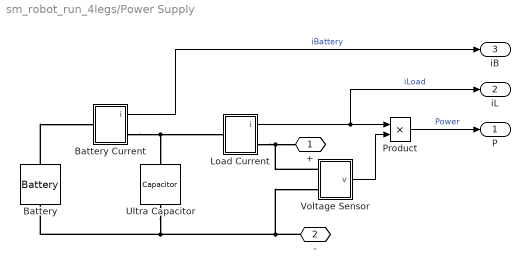
== system sm_robot_run_4legs/Power Supply ==
  Battery : batteryecm_lib/Battery  Vnom=24 V  prm_dir=1  R1_dis=2 Ohm  R1_ch=2 Ohm  R1=1 Ohm  prm_AH=2  AH=10 hr*A  V1=22 V  AH1=5 hr*A  prm_R2=1  R2=2e+03 Ohm  Tmeas=298.15 K  charge_measurement_port=simscape.enum.battery.enable.no  prm_dyn=1  Rp1=0.005 Ohm  tau1=30 s  Rp2=0.005 Ohm  tau2=30 s  Rp3=0.005 Ohm  tau3=30 s  Rp4=0.005 Ohm  tau4=30 s  Rp5=0.005 Ohm  tau5=30 s  prm_fade=1  N_fade=100  AH_fade=45 hr*A  R1_fade=2.02 Ohm  R1_ch_fade=2.02 Ohm  V1_fade=10.35 V  prm_age=1  prm_age_OCV=1  OCV_age=0.9  SOC_age=60  Tmeas_age=298.15 K  delta_time_age_vec=[0] d  temperature_age_vec=[273] K  OCV_scaling_age=2.2134e6  OCV_offset_age=1.632e6  temp_exp_age=0.515833569 V  t_exp_age=0.75  Vnom_T2=12 V  R1_T2=2.2 Ohm  R1_T2_dis=2.2 Ohm  R1_T2_ch=2.2 Ohm  V1_T2=11.4 V  R2_T2=2200 Ohm  Rp1_T2=0.005 Ohm  tau1_T2=30 s  Rp2_T2=0.005 Ohm  tau2_T2=30 s  Rp3_T2=0.005 Ohm  tau3_T2=30 s  Rp4_T2=0.005 Ohm  tau4_T2=30 s  Rp5_T2=0.005 Ohm  tau5_T2=30 s  Tmeas2=273.15 K  thermal_port=simscape.enum.thermaleffects.omit  thermal_mass=30000 J/K  i_specify=off  i_priority=None  i=0 A  i_nominal_specify=off  i_nominal_value=1  i_nominal_unit=A  v_specify=off  v_priority=None  v=0 V  v_nominal_specify=off  v_nominal_value=1  v_nominal_unit=V  charge_specify=on  charge_priority=High  charge=5 hr*A  charge_nominal_specify=off  charge_nominal_value=1  charge_nominal_unit=A*hr  num_cycles_specify=off  num_cycles_priority=High  num_cycles=0  num_cycles_nominal_specify=off  num_cycles_nominal_value=1  num_cycles_nominal_unit=1  temperature_specify=off  temperature_priority=High  temperature=298.15 K  temperature_nominal_specify=off  temperature_nominal_value=1  temperature_nominal_unit=K
  Battery Current : Subsystem
  Load Current : Subsystem
  Product : Product  RndMeth=Zero
  Ultra Capacitor : fl_lib/Electrical/Electrical Elements/Capacitor  c=1 F  r=1e-3 Ohm  g=0 1/Ohm  i_specify=off  i_priority=None  i=0 A  i_nominal_specify=off  i_nominal_value=1  i_nominal_unit=A  v_specify=off  v_priority=None  v=0 V  v_nominal_specify=off  v_nominal_value=1  v_nominal_unit=V  vc_specify=on  vc_priority=High  vc=22 V  vc_nominal_specify=off  vc_nominal_value=1  vc_nominal_unit=V
  Voltage Sensor : Subsystem
  + : PMIOPort  Side=Left
  - : PMIOPort  Port=2  Side=Left
  P : Outport  VectorParamsAs1DForOutWhenUnconnected=off
  iL : Outport  Port=2  VectorParamsAs1DForOutWhenUnconnected=off
  iB : Outport  Port=3  VectorParamsAs1DForOutWhenUnconnected=off
  wires:
  Load Current/1(i) -> iL/1, Product/1  "iLoad"
  Voltage Sensor/1(v) -> Product/2
  Product/1 -> P/1  "Power"
  Battery Current/1(i) -> iB/1  "iBattery"
  connections:
  -/RConn1 -- Voltage Sensor/LConn2 -- Battery/RConn1 -- Ultra Capacitor/RConn1
  Voltage Sensor/LConn1 -- +/RConn1 -- Load Current/RConn1
  Battery/LConn1 -- Battery Current/LConn1
  Battery Current/RConn1 -- Load Current/LConn1 -- Ultra Capacitor/LConn1

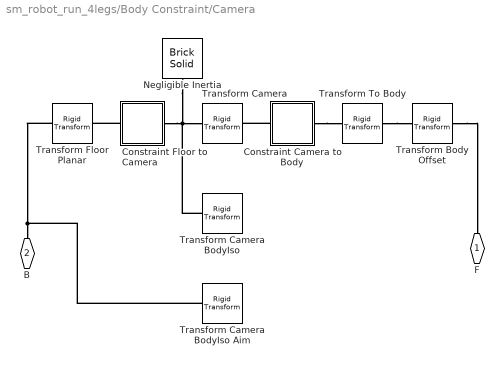
== system sm_robot_run_4legs/Body Constraint/Camera ==
  Constraint Camera to Body : Subsystem  Variant=on  VariantControlMode=label  VariantControl=Variant1  LabelModeActiveChoice=Planar
      settings: AttributesFormatString=%<ActiveVariant>
      mask Display: disp(' ');
  Constraint Floor to Camera : Subsystem  Variant=on  VariantControlMode=label  VariantControl=Variant1  LabelModeActiveChoice=Planar
      settings: AttributesFormatString=%<ActiveVariant>
      mask Display: disp(' ')
  Negligible Inertia : sm_lib/Body Elements/Brick Solid  BrickDimensions=[1 1 1]*1e-3  BrickDimensionsUnits=m  ExportEntireGeometry=off  InertiaType=PointMass  BasedOnType=Density  Density=1000  DensityUnits=kg/m^3  Mass=1e-6  MassUnits=kg  CenterOfMass=[0 0 0]  CenterOfMassUnits=m  MomentsOfInertia=[1 1 1]  MomentsOfInertiaUnits=kg*m^2  ProductsOfInertia=[1 1 1]  ProductsOfInertiaUnits=kg*m^2  GraphicType=FromGeometry  MarkerShape=Sphere  MarkerSize=10  GraphicVisPropType=SimpleVisualProperties  GraphicDiffuseColor=[0.5 0.5 0.5]  GraphicOpacity=1.0  GraphicSpecularColor=[0.5 0.5 0.5 1.0]  GraphicAmbientColor=[0.15 0.15 0.15 1.0]  GraphicEmissiveColor=[0.0 0.0 0.0 1.0]  GraphicShininess=75  DoExposeReferenceFrame=on  SerializedFrames=<Frames/>
  Transform Body Offset : sm_lib/Frames and Transforms/Rigid Transform  RotationMethod=None  FollAlignAxisA=+X  BaseAlignAxisA=+Y  FollAlignAxisB=+Y  BaseAlignAxisB=+Z  RotationStandardAxis=+X  RotationAngle=0  RotationAngleUnits=deg  RotationArbitraryAxis=[0 0 1]  RotationSequenceAxes=FollowerAxes  RotationSequence=XYX  RotationSequenceAngles=[0 0 0]  RotationSequenceAnglesUnits=deg  RotationMatrix=[1 0 0; 0 1 0; 0 0 1]  Quaternion=[1 0 0 0]  TranslationMethod=StandardAxis  TranslationCartesianOffset=[0 0 0]  TranslationCartesianOffsetUnits=m  TranslationStandardAxis=-Z  TranslationStandardOffset=2  TranslationStandardOffsetUnits=m  TranslationROffset=0  TranslationROffsetUnits=m  TranslationThetaOffset=0  TranslationThetaOffsetUnits=deg  TranslationZOffset=0  TranslationZOffsetUnits=m
  Transform Camera : sm_lib/Frames and Transforms/Rigid Transform  RotationMethod=None  FollAlignAxisA=+X  BaseAlignAxisA=+Y  FollAlignAxisB=+Y  BaseAlignAxisB=+Z  RotationStandardAxis=+Z  RotationAngle=0.0  RotationAngleUnits=deg  RotationArbitraryAxis=[0 0 1]  RotationSequenceAxes=FollowerAxes  RotationSequence=XYX  RotationSequenceAngles=[0 0 0]  RotationSequenceAnglesUnits=deg  RotationMatrix=[1 0 0; 0 1 0; 0 0 1]  Quaternion=[1 0 0 0]  TranslationMethod=StandardAxis  TranslationCartesianOffset=[0 0 0]  TranslationCartesianOffsetUnits=m  TranslationStandardAxis=+Z  TranslationStandardOffset=L_stance/2  TranslationStandardOffsetUnits=m  TranslationROffset=0  TranslationROffsetUnits=m  TranslationThetaOffset=0  TranslationThetaOffsetUnits=deg  TranslationZOffset=0  TranslationZOffsetUnits=m
  Transform Camera BodyIso : sm_lib/Frames and Transforms/Rigid Transform  RotationMethod=None  FollAlignAxisA=+X  BaseAlignAxisA=+Y  FollAlignAxisB=+Y  BaseAlignAxisB=+Z  RotationStandardAxis=+Z  RotationAngle=0.0  RotationAngleUnits=deg  RotationArbitraryAxis=[0 0 1]  RotationSequenceAxes=FollowerAxes  RotationSequence=XYX  RotationSequenceAngles=[0 0 0]  RotationSequenceAnglesUnits=deg  RotationMatrix=[1 0 0; 0 1 0; 0 0 1]  Quaternion=[1 0 0 0]  TranslationMethod=Cartesian  TranslationCartesianOffset=[2.5 0.8+0.2 L_stance*1.1]  TranslationCartesianOffsetUnits=m  TranslationStandardAxis=+Z  TranslationStandardOffset=0  TranslationStandardOffsetUnits=m  TranslationROffset=0  TranslationROffsetUnits=m  TranslationThetaOffset=0  TranslationThetaOffsetUnits=deg  TranslationZOffset=0  TranslationZOffsetUnits=m
  Transform Camera BodyIso Aim : sm_lib/Frames and Transforms/Rigid Transform  RotationMethod=RotationSequence  FollAlignAxisA=+X  BaseAlignAxisA=+Y  FollAlignAxisB=+Y  BaseAlignAxisB=+Z  RotationStandardAxis=+Y  RotationAngle=60  RotationAngleUnits=deg  RotationArbitraryAxis=[0 0 1]  RotationSequenceAxes=FollowerAxes  RotationSequence=YXY  RotationSequenceAngles=[60 -10 0]  RotationSequenceAnglesUnits=deg  RotationMatrix=[1 0 0; 0 1 0; 0 0 1]  Quaternion=[1 0 0 0]  TranslationMethod=Cartesian  TranslationCartesianOffset=[1 1 L_stance/2]  TranslationCartesianOffsetUnits=m  TranslationStandardAxis=+Z  TranslationStandardOffset=0  TranslationStandardOffsetUnits=m  TranslationROffset=0  TranslationROffsetUnits=m  TranslationThetaOffset=0  TranslationThetaOffsetUnits=deg  TranslationZOffset=0  TranslationZOffsetUnits=m
  Transform Floor Planar : sm_lib/Frames and Transforms/Rigid Transform  RotationMethod=StandardAxis  FollAlignAxisA=+X  BaseAlignAxisA=+Y  FollAlignAxisB=+Y  BaseAlignAxisB=+Z  RotationStandardAxis=-X  RotationAngle=90  RotationAngleUnits=deg  RotationArbitraryAxis=[0 0 1]  RotationSequenceAxes=FollowerAxes  RotationSequence=XYX  RotationSequenceAngles=[0 0 0]  RotationSequenceAnglesUnits=deg  RotationMatrix=[1 0 0; 0 1 0; 0 0 1]  Quaternion=[1 0 0 0]  TranslationMethod=None  TranslationCartesianOffset=[0 0 0]  TranslationCartesianOffsetUnits=m  TranslationStandardAxis=+Z  TranslationStandardOffset=0  TranslationStandardOffsetUnits=m  TranslationROffset=0  TranslationROffsetUnits=m  TranslationThetaOffset=0  TranslationThetaOffsetUnits=deg  TranslationZOffset=0  TranslationZOffsetUnits=m
  Transform To Body : sm_lib/Frames and Transforms/Rigid Transform  RotationMethod=StandardAxis  FollAlignAxisA=+X  BaseAlignAxisA=+Y  FollAlignAxisB=+Y  BaseAlignAxisB=+Z  RotationStandardAxis=+X  RotationAngle=90  RotationAngleUnits=deg  RotationArbitraryAxis=[0 0 1]  RotationSequenceAxes=FollowerAxes  RotationSequence=XYX  RotationSequenceAngles=[0 0 0]  RotationSequenceAnglesUnits=deg  RotationMatrix=[1 0 0; 0 1 0; 0 0 1]  Quaternion=[1 0 0 0]  TranslationMethod=None  TranslationCartesianOffset=[0 0 0]  TranslationCartesianOffsetUnits=m  TranslationStandardAxis=+Z  TranslationStandardOffset=0  TranslationStandardOffsetUnits=m  TranslationROffset=0  TranslationROffsetUnits=m  TranslationThetaOffset=0  TranslationThetaOffsetUnits=deg  TranslationZOffset=0  TranslationZOffsetUnits=m
  F : PMIOPort  Side=Right
  B : PMIOPort  Port=2  Side=Left
  connections:
  Transform Floor Planar/LConn1 -- Transform Camera BodyIso Aim/LConn1 -- B/RConn1
  Transform To Body/RConn1 -- Transform Body Offset/LConn1
  Transform Body Offset/RConn1 -- F/RConn1
  Negligible Inertia/RConn1 -- Transform Camera BodyIso/LConn1 -- Constraint Floor to Camera/RConn1 -- Transform Camera/LConn1
  Constraint Floor to Camera/LConn1 -- Transform Floor Planar/RConn1
  Constraint Camera to Body/LConn1 -- Transform Camera/RConn1
  Constraint Camera to Body/RConn1 -- Transform To Body/LConn1

== system sm_robot_run_4legs/Body Constraint/Constraint ==
  Planar : Subsystem  VariantControl=Planar
  Six DOF : Subsystem  VariantControl=Six_DOF
  " B " : PMIOPort  Side=Left
  " F " : PMIOPort  Port=2  Side=Right

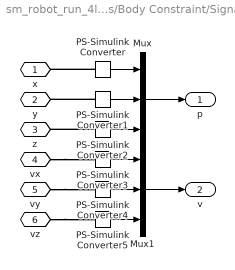
== system sm_robot_run_4legs/Body Constraint/Signals ==
  Mux : Mux  Inputs=3
  Mux1 : Mux  Inputs=3
  PS-Simulink Converter{,1..5} (6 alike) : nesl_utility/PS-Simulink Converter  PhysicalDomain=network_engine_domain  SubClassName=ps_output  LeftPortType=input  RightPortType=output  PseudoPeriodic=off  Frequencies=[]  VectorFormat=1-D array  Unit=1  AffineConversion=off
  x : PMIOPort  Side=Left
  y : PMIOPort  Port=2  Side=Left
  z : PMIOPort  Port=3  Side=Left
  vx : PMIOPort  Port=4  Side=Left
  vy : PMIOPort  Port=5  Side=Left
  vz : PMIOPort  Port=6  Side=Left
  p : Outport  VectorParamsAs1DForOutWhenUnconnected=off
  v : Outport  Port=2  VectorParamsAs1DForOutWhenUnconnected=off
  wires:
  Mux/1 -> p/1
  PS-Simulink Converter1/1 -> Mux/2
  PS-Simulink Converter2/1 -> Mux/3
  PS-Simulink Converter/1 -> Mux/1
  PS-Simulink Converter4/1 -> Mux1/2
  PS-Simulink Converter5/1 -> Mux1/3
  Mux1/1 -> v/1
  PS-Simulink Converter3/1 -> Mux1/1
  connections:
  PS-Simulink Converter1/LConn1 -- y/RConn1
  PS-Simulink Converter/LConn1 -- x/RConn1
  vz/RConn1 -- PS-Simulink Converter5/LConn1
  vx/RConn1 -- PS-Simulink Converter3/LConn1
  vy/RConn1 -- PS-Simulink Converter4/LConn1
  PS-Simulink Converter2/LConn1 -- z/RConn1

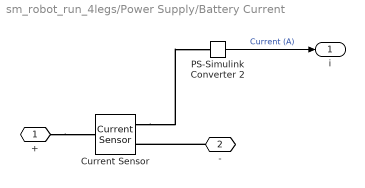
== system sm_robot_run_4legs/Power Supply/Battery Current ==
  Current Sensor : fl_lib/Electrical/Electrical Sensors/Current Sensor
  PS-Simulink Converter 2 : nesl_utility/PS-Simulink Converter  PhysicalDomain=network_engine_domain  SubClassName=ps_output  LeftPortType=input  RightPortType=output  PseudoPeriodic=off  Frequencies=[]  VectorFormat=1-D array  Unit=A  AffineConversion=off
  + : PMIOPort  Side=Left
  - : PMIOPort  Port=2  Side=Right
  i : Outport  VectorParamsAs1DForOutWhenUnconnected=off
  wires:
  PS-Simulink Converter 2/1 -> i/1  "Current (A)"
  connections:
  +/RConn1 -- Current Sensor/LConn1
  -/RConn1 -- Current Sensor/RConn2
  Current Sensor/RConn1 -- PS-Simulink Converter 2/LConn1

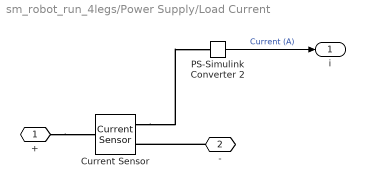
== system sm_robot_run_4legs/Power Supply/Load Current ==
  Current Sensor : fl_lib/Electrical/Electrical Sensors/Current Sensor
  PS-Simulink Converter 2 : nesl_utility/PS-Simulink Converter  PhysicalDomain=network_engine_domain  SubClassName=ps_output  LeftPortType=input  RightPortType=output  PseudoPeriodic=off  Frequencies=[]  VectorFormat=1-D array  Unit=A  AffineConversion=off
  + : PMIOPort  Side=Left
  - : PMIOPort  Port=2  Side=Right
  i : Outport  VectorParamsAs1DForOutWhenUnconnected=off
  wires:
  PS-Simulink Converter 2/1 -> i/1  "Current (A)"
  connections:
  Current Sensor/RConn1 -- PS-Simulink Converter 2/LConn1
  -/RConn1 -- Current Sensor/RConn2
  +/RConn1 -- Current Sensor/LConn1

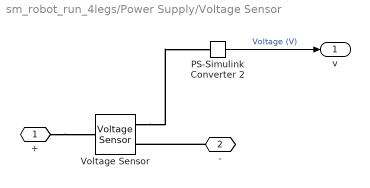
== system sm_robot_run_4legs/Power Supply/Voltage Sensor ==
  PS-Simulink Converter 2 : nesl_utility/PS-Simulink Converter  PhysicalDomain=network_engine_domain  SubClassName=ps_output  LeftPortType=input  RightPortType=output  PseudoPeriodic=off  Frequencies=[]  VectorFormat=1-D array  Unit=V  AffineConversion=off
  Voltage Sensor : fl_lib/Electrical/Electrical Sensors/Voltage Sensor
  + : PMIOPort  Side=Left
  - : PMIOPort  Port=2  Side=Left
  v : Outport  VectorParamsAs1DForOutWhenUnconnected=off
  wires:
  PS-Simulink Converter 2/1 -> v/1  "Voltage (V)"
  connections:
  +/RConn1 -- Voltage Sensor/LConn1
  -/RConn1 -- Voltage Sensor/RConn2
  Voltage Sensor/RConn1 -- PS-Simulink Converter 2/LConn1

== system sm_robot_run_4legs/Body Constraint/Camera/Constraint Camera to Body ==
  Planar : Subsystem  VariantControl=Planar
  SixDOF : Subsystem  VariantControl=Six_DOF
  " B " : PMIOPort  Side=Left
  " F " : PMIOPort  Port=2  Side=Right

== system sm_robot_run_4legs/Body Constraint/Camera/Constraint Floor to Camera ==
  Planar : Subsystem  VariantControl=Planar
  SixDOF : Subsystem  VariantControl=Six_DOF
  " B " : PMIOPort  Side=Left
  " F " : PMIOPort  Port=2  Side=Right
